simulink model "furuta_pi_function_check"  (R2026b)
settings: Solver=FixedStepDiscrete  StopTime=.05  FixedStep=.01
settings Model: Creator=Lsh  LastModifiedBy=Lsh

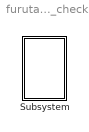
== system furuta_pi_function_check ==
  Subsystem : Subsystem

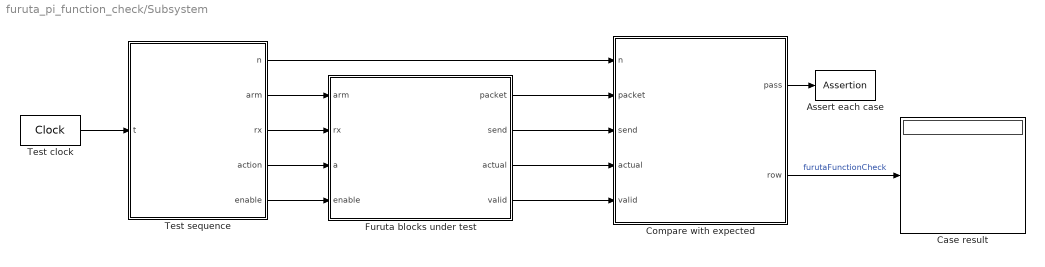
== system furuta_pi_function_check/Subsystem ==
  Assert each case : Assertion
  Case result : Display
  Compare with expected : MATLAB Function  TreatAsAtomicUnit=on
  Furuta blocks under test : MATLAB Function  TreatAsAtomicUnit=on
  Test clock : DigitalClock  SampleTime=.01
  Test sequence : MATLAB Function  TreatAsAtomicUnit=on
  wires:
  Test sequence/4(action) -> Furuta blocks under test/3(a)
  Test sequence/3(rx) -> Furuta blocks under test/2(rx)
  Test sequence/1(n) -> Compare with expected/1(n)
  Compare with expected/1(pass) -> Assert each case/1
  Furuta blocks under test/1(packet) -> Compare with expected/2(packet)
  Test clock/1 -> Test sequence/1(t)
  Test sequence/2(arm) -> Furuta blocks under test/1(arm)
  Furuta blocks under test/2(send) -> Compare with expected/3(send)
  Furuta blocks under test/3(actual) -> Compare with expected/4(actual)
  Compare with expected/2(row) -> Case result/1  "furutaFunctionCheck"
  Test sequence/5(enable) -> Furuta blocks under test/4(enable)
  Furuta blocks under test/4(valid) -> Compare with expected/5(valid)

== matlab function furuta_pi_function_check/Subsystem/Furuta blocks under test ==
  data: arm input; packet output; rx input; a input; enable input; send output; actual output; valid output
function [packet,send,actual,valid] = test(arm,rx,a,enable)
[o,valid] = furuta_pi_decode(arm,rx,uint8(32),uint8([15 219]),[-209.05 -1 4058.5 1],.01);
[packet,send,actual] = furuta_pi_frame(a,o,valid,enable,1,1,.1,ones(1,4),0,1);
end

== matlab function furuta_pi_function_check/Subsystem/Test sequence ==
  data: t input; n output; arm output; rx output; action output; enable output
function [n,arm,rx,action,enable] = cases(t)
n = min(5,round(t/.01));
arm = uint8([146 0 0 0 87 174 255 255]);
rx = n~=3;
action = 1-2*double(n==2);
enable = n~=0;
end

== matlab function furuta_pi_function_check/Subsystem/Compare with expected ==
  data: n input; pass output; packet input; send input; actual input; valid input; row output
function [pass,row] = compare(n,packet,send,actual,valid)
expectedOpcode = uint8([0 161 161 128 128 128]);
expectedLow = uint8([0 10 246 0 0 0]);
expectedHigh = uint8([0 0 255 0 0 0]);
expectedAction = [0 .1 -.1 0 0 0];
expectedValid = [false true true false false true];
i = n+1;
expected = [expectedOpcode(i) 0 0 0 expectedLow(i) expectedHigh(i) 0 0];
pass = all(packet==expected) && send==(n~=0) && actual==expectedAction(i) && valid==expectedValid(i);
row = [n;double(pass);double(packet(1));actual;double(valid)];
end
